simulink model "SolarTrackingModel"  (R2022b)
settings: Solver=FixedStepAuto  StartTime=0.0  StopTime=50  RelTol=1e-3  EnableMultiTasking=on
libraries: SignalEditorBlockLib x3
settings Model: ExtModeTrigDuration=2  Creator=ASUS  LastModifiedBy=LENOVO
settings OptimizationCC: DefaultParameterBehavior=Inlined  EnhancedBackFolding=on  PassReuseOutputArgsAs=Individual arguments  ZeroExternalMemoryAtStartup=off  ZeroInternalMemoryAtStartup=off  MaxStackSize=64  OptimizeBlockOrder=speed  DifferentSizesBufferReuse=on  OptimizationCustomize=off  EfficientTunableParamExpr=on
settings DebuggingCC: ParameterTunabilityLossMsg=error  UnconnectedInputMsg=warning  UnconnectedOutputMsg=warning  UnconnectedLineMsg=warning  SFInvalidInputDataAccessInChartInitDiag=error
settings HardwareCC: ProdBitPerInt=16  ProdBitPerPointer=16  ProdBitPerSizeT=16  ProdBitPerPtrDiffT=16  ProdLargestAtomicFloat=None  ProdWordSize=8  ProdHWDeviceType=Atmel->AVR
settings ModelReferenceCC: EnableRefExpFcnMdlSchedulingChecks=on
settings SFSimCC: MATLABDynamicMemAlloc=off
settings RTWCC: Description=Embedded Coder  SystemTargetFile=ert.tlc  HardwareBoard=Arduino Uno  TLCOptions=-aInlineSetEventsForThisBaseRateFcn=TLC_FALSE -aSuppressMultiTaskScheduler=TLC_FALSE -aRateBasedStepFcn=1  TemplateMakefile=ert_default_tmf  GenerateReport=on  Toolchain=Arduino AVR  BuildConfiguration=Faster Runs  LaunchReport=on  DLArmComputeVersion=19.05
settings CodeAppCC: ForceParamTrailComments=on  IgnoreCustomStorageClasses=off  OperatorAnnotations=on  SimulinkDataObjDesc=on  SFDataObjDesc=on  InsertBlockDesc=on
settings ERTTargetCC: UtilityFuncGeneration=Shared location  CombineSignalStateStructs=on  SuppressErrorStatus=on  ExtModeTransport=3  ExtModeStaticAlloc=on  ExtModeAutomaticAllocSize=off  ExtModeStaticAllocSize=250  ExtModeMexFile=ext_xcp  ExtModeIntrfLevel=Level2 - Open  InlinedParameterPlacement=NonHierarchical

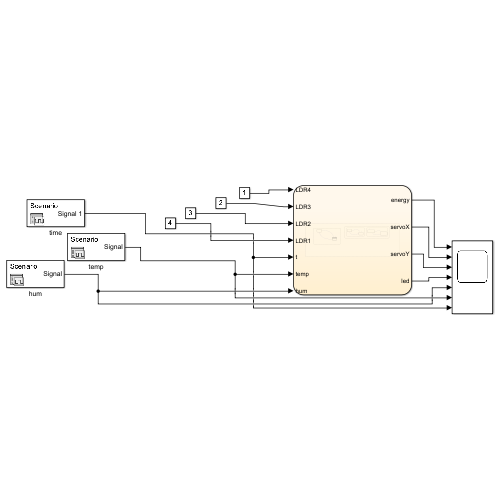
[thumbnail: Simulink's stored preview of the top-level diagram]
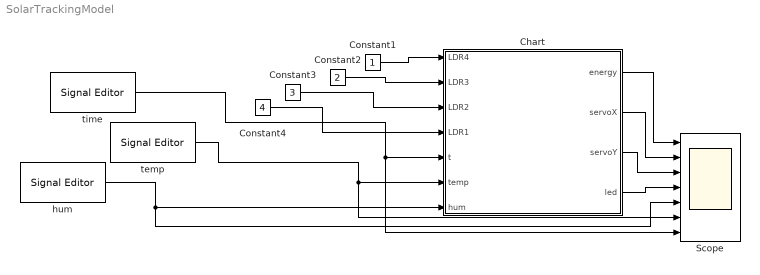
== system SolarTrackingModel ==
  Chart : Stateflow chart  TreatAsAtomicUnit=on
  Constant1 : Constant
  Constant2 : Constant  Value=2
  Constant3 : Constant  Value=3
  Constant4 : Constant  Value=4
  Scope : Scope  NumInputPorts=7
  hum : SignalEditorBlockLib/Signal Editor  FileName=humidity.mat  ActiveScenario=Scenario  ActiveSignal=Signal  IsBus=off  OutputBusObjectStr=Bus: BusObject  SampleTime=0  Interpolate=off  ZeroCross=off  OutputAfterFinalValue=Setting to zero  Unit=inherit  PreserveSignalName=on
  temp : SignalEditorBlockLib/Signal Editor  FileName=humidity.mat  ActiveScenario=Scenario  ActiveSignal=Signal  IsBus=off  OutputBusObjectStr=Bus: BusObject  SampleTime=0  Interpolate=off  ZeroCross=off  OutputAfterFinalValue=Setting to zero  Unit=inherit  PreserveSignalName=on
  time : SignalEditorBlockLib/Signal Editor  FileName=time.mat  ActiveScenario=Scenario  ActiveSignal=Signal 1  IsBus=off  OutputBusObjectStr=Bus: BusObject  SampleTime=0  Interpolate=off  ZeroCross=off  OutputAfterFinalValue=Setting to zero  Unit=inherit  PreserveSignalName=on
  wires:
  Constant1/1 -> Chart/1(LDR4)
  Constant2/1 -> Chart/2(LDR3)
  Constant3/1 -> Chart/3(LDR2)
  Constant4/1 -> Chart/4(LDR1)
  Chart/1(energy) -> Scope/1
  Chart/2(servoX) -> Scope/2
  Chart/3(servoY) -> Scope/3
  hum/1 -> Scope/5, Chart/7(hum)
  temp/1 -> Scope/6, Chart/6(temp)
  time/1 -> Scope/7, Chart/5(t)
  Chart/4(led) -> Scope/4

== stateflow chart SolarTrackingModel/Chart ==
  state PowerOn [parallel]
    settings: executionOrder=1
    state EnergyManagement [parallel]
      settings: executionOrder=1
      state EnergyLevel [parallel]
        settings: executionOrder=2
        state LowEnergy
          led = 1;
        state Normal
          led = 0;
        LowEnergy -> Normal : [energy >=20]
        (default) -> Normal
        Normal -> LowEnergy : [energy < 20]
      state DailyCycle [parallel]
        settings: executionOrder=1
        state Day
          energy = min(energy + 10, 100);
        state Night
          energy = max(energy / 1.3, 0);
        (default) -> Day
        Day -> Night : [t < 0]
        Night -> Day : [t >= 0]
    state EnvMonitoring [parallel]
      settings: executionOrder=2
      state Danger
        servoX = 90;
        servoY = 90;
      state Safe
        state MoveRight
          servoX = servoX + 1;
        state MoveLeft
          servoX = servoX - 1;
        state Idle
        state MoveUp
          servoY = servoY +1;
        state MoveDown
          servoY = servoY -1;
        MoveRight -> Idle : [(LDR4 <= LDR2) | (LDR4 <= LDR3) | (LDR4 <= LDR1)]
        MoveLeft -> Idle : [(LDR2 <= LDR1) | (LDR2 <= LDR3) | (LDR2 <= LDR4)]
        Idle -> MoveRight [order 1] : [(LDR4> LDR1) & (LDR4 > LDR2) & (LDR4 > LDR3)]
        Idle -> MoveLeft [order 2] : [(LDR2 > LDR1) & (LDR2 > LDR3) & (LDR2 > LDR4)]
        (default) -> Idle
        MoveDown -> Idle : [(LDR3 <= LDR2) | (LDR3 <= LDR1) | (LDR3 <= LDR4)]
        MoveUp -> Idle : [(LDR1 <= LDR2) | (LDR1 <= LDR3) | (LDR1 <= LDR4)]
        Idle -> MoveUp [order 3] : [(LDR1 > LDR2) & (LDR1 > LDR3) & (LDR1 > LDR4)]
        Idle -> MoveDown [order 4] : [(LDR3 > LDR1) & (LDR3 > LDR2) & (LDR3 > LDR4)]
      Danger -> Safe : [(temp <= 40 && hum <= 80)]
      Safe -> Danger : [(temp > 40 || hum > 80)]
      (default) -> Safe
  data: LDR4 input; LDR3 input; LDR2 input; energy output =1; servoX output =0; LDR1 input; t input; servoY output =0; led output =0; temp input; hum input
